simulink model "DT4H_SIMULATION_EEE"  (R2025b)
settings: Solver=ode3  StartTime=0.0  StopTime=10.0  RelTol=1e-3
libraries: simulink x19, dspstat3 x6, fuzblock x1
(part 1 of 3)
settings Model: Creator=harsh  LastModifiedBy=harsh

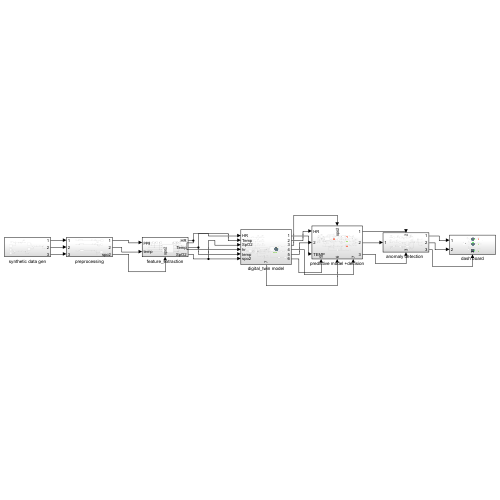
[thumbnail: Simulink's stored preview of the top-level diagram]
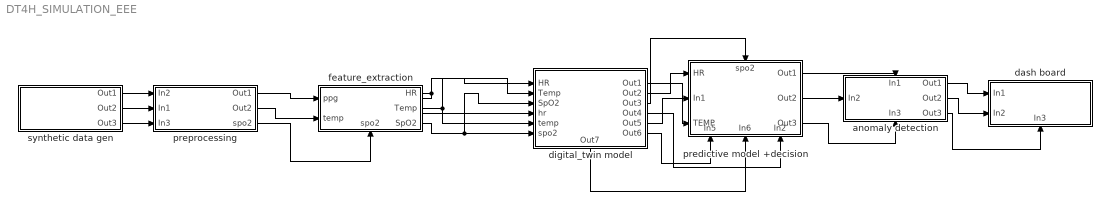
== system DT4H_SIMULATION_EEE ==
  "anomaly detection  " : Subsystem
      settings: PortSchema="{\"entries\":[{\"content\":{\"sides\":[{\"content\":{\"connectorIds\":[\"In1\"]},\"type\":\"ConnectorPlacement.EquallySpacedRectSide\",\"uuid\":\"25253e62-3c40-49ae-b2f5-e9d5db3c8bc6\"},{\"content\":{\"connectorIds\":[\"Out1\",\"Out2\",\"Out3\"],\"side\":\"RIGHT\"},\"type\":\"ConnectorPlacement.EquallySpacedRectSide\",\"uuid\":\"f4a70f19-11e9-4566-a749-a521162cf708\"},{\"content\":{\"connectorIds\":[\"In2\"],\"side\":\"TOP\"},\"type\":\"ConnectorPlacement.EquallySpacedRectSide\",\"uuid\":\"d5382edc-197f-43a2-9fdd-3d2ad96da76a\"},{\"content\":{\"connectorIds\":[\"In3\"],\"side\":\"BOTTOM\"},\"type\":\"ConnectorPlacement.EquallySpacedRectSide\",\"uuid\":\"cc34089e-1bbc-443e-9edf-3f88c550613d\"}]},\"type\":\"ConnectorPlacement.EquallySpacedConnector\",\"uuid\":\"d18f1512-da4b-4774-865f-899ab03939b9\"}],\"packageUris\":[\"http://schema.mathworks.com/mf0/Connector/R2020b\"],\"version\":\"1.0\"}"
  dash board : Subsystem
      settings: PortSchema="{\"entries\":[{\"content\":{\"sides\":[{\"content\":{\"connectorIds\":[\"In1\",\"In2\"]},\"type\":\"ConnectorPlacement.EquallySpacedRectSide\",\"uuid\":\"cdd0eb8c-e2f0-4f49-b522-7982e33a9b2a\"},{\"content\":{\"side\":\"RIGHT\"},\"type\":\"ConnectorPlacement.EquallySpacedRectSide\",\"uuid\":\"02186336-f3a8-4644-896c-78cbe002086a\"},{\"content\":{\"side\":\"TOP\"},\"type\":\"ConnectorPlacement.EquallySpacedRectSide\",\"uuid\":\"908a15e8-0b5f-4f2f-82b4-ba6efd9ebe98\"},{\"content\":{\"connectorIds\":[\"In3\"],\"side\":\"BOTTOM\"},\"type\":\"ConnectorPlacement.EquallySpacedRectSide\",\"uuid\":\"1bb7e8d6-76d1-4f36-b622-8394fe1e0f54\"}]},\"type\":\"ConnectorPlacement.EquallySpacedConnector\",\"uuid\":\"3009d2cf-5250-4716-8b2f-345bda64d323\"}],\"packageUris\":[\"http://schema.mathworks.com/mf0/Connector/R2020b\"],\"version\":\"1.0\"}"
  digital_twin model : Subsystem
      settings: PortSchema="{\"entries\":[{\"content\":{\"sides\":[{\"content\":{\"connectorIds\":[\"In1\",\"In2\",\"In3\",\"In4\",\"In5\",\"In6\"]},\"type\":\"ConnectorPlacement.EquallySpacedRectSide\",\"uuid\":\"60b3441d-3906-42cd-a64f-c568a4e10bef\"},{\"content\":{\"connectorIds\":[\"Out1\",\"Out2\",\"Out3\",\"Out4\",\"Out5\",\"Out6\"],\"side\":\"RIGHT\"},\"type\":\"ConnectorPlacement.EquallySpacedRectSide\",\"uuid\":\"87df974d-96fc-4f5d-987f-b85e09fb9cb4\"},{\"content\":{\"side\":\"TOP\"},\"type\":\"ConnectorPlacement.EquallySpacedRectSide\",\"uuid\":\"bcc1c708-069a-4209-9e3d-4d3f31c3ddac\"},{\"content\":{\"connectorIds\":[\"Out7\"],\"side\":\"BOTTOM\"},\"type\":\"ConnectorPlacement.EquallySpacedRectSide\",\"uuid\":\"6497df40-0368-42cc-9f26-60ecc793cf19\"}]},\"type\":\"ConnectorPlacement.EquallySpacedConnector\",\"uuid\":\"1b248ab8-3cfb-4c5b-9a5f-89bd9e36bb2e\"}],\"packageUris\":[\"http://schema.mathworks.com/mf0/Connector/R2020b\"],\"version\":\"1.0\"}"
  feature_extraction : Subsystem
      settings: PortSchema="{\"entries\":[{\"content\":{\"sides\":[{\"content\":{\"connectorIds\":[\"In1\",\"In2\"]},\"type\":\"ConnectorPlacement.EquallySpacedRectSide\",\"uuid\":\"0c4b2ed4-113f-4166-b962-4d2c86f0b3f8\"},{\"content\":{\"connectorIds\":[\"Out1\",\"Out2\",\"Out3\"],\"side\":\"RIGHT\"},\"type\":\"ConnectorPlacement.EquallySpacedRectSide\",\"uuid\":\"e3832425-a364-440c-8c10-9734fc320651\"},{\"content\":{\"side\":\"TOP\"},\"type\":\"ConnectorPlacement.EquallySpacedRectSide\",\"uuid\":\"36c7fb6d-317e-4b4f-ae9e-aa12a7efa738\"},{\"content\":{\"connectorIds\":[\"In3\"],\"side\":\"BOTTOM\"},\"type\":\"ConnectorPlacement.EquallySpacedRectSide\",\"uuid\":\"d821c285-c54e-4db5-b1a8-90f41e6ccbda\"}]},\"type\":\"ConnectorPlacement.EquallySpacedConnector\",\"uuid\":\"1bb0afcd-9a28-4be8-abf5-d992c306dad6\"}],\"packageUris\":[\"http://schema.mathworks.com/mf0/Connector/R2020b\"],\"version\":\"1.0\"}"
  predictive model +decision : Subsystem
      settings: PortSchema="{\"entries\":[{\"content\":{\"sides\":[{\"content\":{\"connectorIds\":[\"In1\",\"In2\",\"In3\"]},\"type\":\"ConnectorPlacement.EquallySpacedRectSide\",\"uuid\":\"b7d4fdfc-ed91-464e-87ae-7c928519d529\"},{\"content\":{\"connectorIds\":[\"Out1\",\"Out2\",\"Out3\"],\"side\":\"RIGHT\"},\"type\":\"ConnectorPlacement.EquallySpacedRectSide\",\"uuid\":\"11799bdd-7268-4954-a90f-71333eb12373\"},{\"content\":{\"connectorIds\":[\"In4\"],\"side\":\"TOP\"},\"type\":\"ConnectorPlacement.EquallySpacedRectSide\",\"uuid\":\"f3428630-4ced-4085-ba1c-f5b921f7daca\"},{\"content\":{\"connectorIds\":[\"In5\",\"In6\",\"In7\"],\"side\":\"BOTTOM\"},\"type\":\"ConnectorPlacement.EquallySpacedRectSide\",\"uuid\":\"6bf4046d-5d73-4edf-8fc4-5c2e0fba2535\"}]},\"type\":\"ConnectorPlacement.EquallySpacedConnector\",\"uuid\":\"07f606c2-3e00-4eb2-b545-ac31073d3b11\"}],\"packageUris\":[\"http://schema.mathworks.com/mf0/Connector/R2020b\"],\"version\":\"1.0\"}"
  preprocessing : Subsystem
  synthetic data gen : Subsystem
  wires:
  feature_extraction/3(SpO2) -> digital_twin model/3(SpO2), digital_twin model/6(spo2)
  digital_twin model/6(Out6) -> predictive model +decision/5(In5)
  "anomaly detection  "/2(Out2) -> dash board/2(In2)
  predictive model +decision/3(Out3) -> "anomaly detection  "/3(In3)
  feature_extraction/2(Temp) -> digital_twin model/5(temp), digital_twin model/2(Temp)
  digital_twin model/2(Out2) -> predictive model +decision/1(HR)
  preprocessing/3(spo2) -> feature_extraction/3(spo2)
  digital_twin model/3(Out3) -> predictive model +decision/4(spo2)
  digital_twin model/1(Out1) -> predictive model +decision/3(TEMP)
  digital_twin model/4(Out4) -> predictive model +decision/7(In2)
  synthetic data gen/1(Out1) -> preprocessing/1(In2)
  "anomaly detection  "/1(Out1) -> dash board/1(In1)
  predictive model +decision/1(Out1) -> "anomaly detection  "/2(In1)
  synthetic data gen/3(Out3) -> preprocessing/3(In3)
  preprocessing/1(Out1) -> feature_extraction/1(ppg)
  predictive model +decision/2(Out2) -> "anomaly detection  "/1(In2)
  digital_twin model/5(Out5) -> predictive model +decision/2(In1)
  feature_extraction/1(HR) -> digital_twin model/4(hr), digital_twin model/1(HR)
  "anomaly detection  "/3(Out3) -> dash board/3(In3)
  digital_twin model/7(Out7) -> predictive model +decision/6(In6)
  preprocessing/2(Out2) -> feature_extraction/2(temp)
  synthetic data gen/2(Out2) -> preprocessing/2(In1)

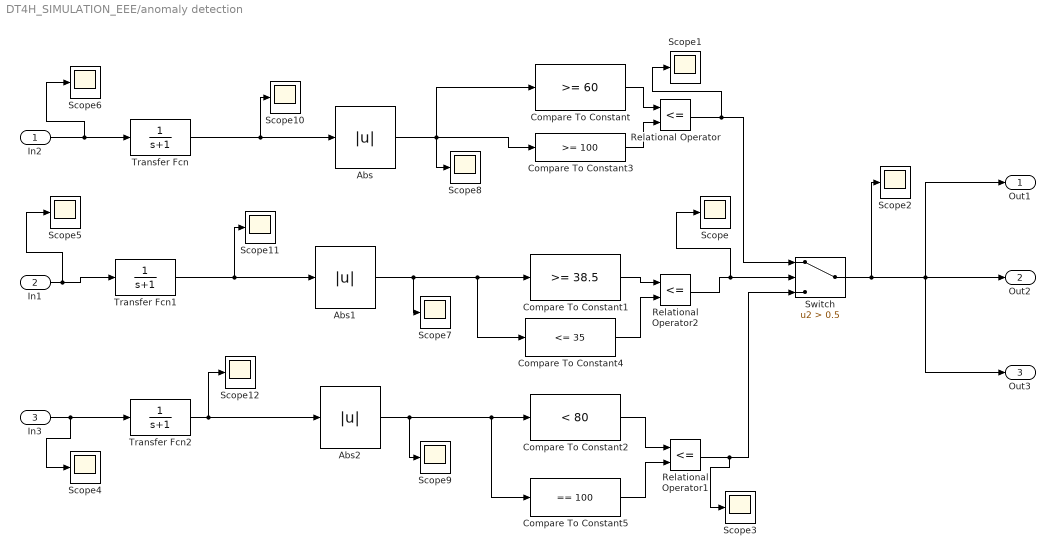
== system DT4H_SIMULATION_EEE/anomaly detection   ==
  In2 : Inport
  In1 : Inport  Port=2
  In3 : Inport  Port=3
  Abs : Abs  SaturateOnIntegerOverflow=off
  Abs1 : Abs  SaturateOnIntegerOverflow=off
  Abs2 : Abs  SaturateOnIntegerOverflow=off
  Compare To Constant : simulink/Logic and Bit Operations/Compare To Constant  relop=>=  const=60  OutDataTypeStr=boolean
  Compare To Constant1 : simulink/Logic and Bit Operations/Compare To Constant  relop=>=  const=38.5  OutDataTypeStr=boolean
  Compare To Constant2 : simulink/Logic and Bit Operations/Compare To Constant  relop=<  const=80  OutDataTypeStr=boolean
  Compare To Constant3 : simulink/Logic and Bit Operations/Compare To Constant  relop=>=  const=100  OutDataTypeStr=boolean
  Compare To Constant4 : simulink/Logic and Bit Operations/Compare To Constant  relop=<=  const=35  OutDataTypeStr=boolean
  Compare To Constant5 : simulink/Logic and Bit Operations/Compare To Constant  relop===  const=100  OutDataTypeStr=boolean
  Relational Operator : RelationalOperator  Operator=<=  OutDataTypeStr=boolean  RndMeth=Simplest  InputSameDT=off
  Relational Operator1 : RelationalOperator  Operator=<=  OutDataTypeStr=boolean  RndMeth=Simplest  InputSameDT=off
  Relational Operator2 : RelationalOperator  Operator=<=  OutDataTypeStr=boolean  RndMeth=Simplest  InputSameDT=off
  Scope{,1..12} (13 alike) : Scope
      Scope settings: ActiveDisplayYMinimum=-0.1649767287234043  ActiveDisplayYMaximum=1.1475232712765957  DataLoggingVariableName=ScopeData35  DataLoggingSaveFormat=Array
      Scope1 settings: ActiveDisplayYMinimum=-1.3578393063829792  ActiveDisplayYMaximum=1.4563615389295217  DataLoggingVariableName=ScopeData36  DataLoggingSaveFormat=Array
      Scope10 settings: ActiveDisplayYMinimum=-0.48272800637728419  ActiveDisplayYMaximum=1.3640066102669111  DataLoggingVariableName=ScopeData45  DataLoggingSaveFormat=Array
      Scope11 settings: ActiveDisplayYMinimum=-1  ActiveDisplayYMaximum=1  DataLoggingVariableName=ScopeData46  DataLoggingSaveFormat=Array
      Scope12 settings: ActiveDisplayYMinimum=-1  ActiveDisplayYMaximum=1  DataLoggingVariableName=ScopeData47  DataLoggingSaveFormat=Array
      Scope2 settings: ActiveDisplayYMinimum=-0.61808118008886315  ActiveDisplayYMaximum=1.4180371033829395  DataLoggingVariableName=ScopeData37  DataLoggingSaveFormat=Array
      Scope3 settings: ActiveDisplayYMinimum=-0.28820857928494759  ActiveDisplayYMaximum=0.38906240889493249  DataLoggingVariableName=ScopeData38  DataLoggingSaveFormat=Array
      Scope4 settings: DataLoggingVariableName=ScopeData39  DataLoggingSaveFormat=Array
      Scope5 settings: ActiveDisplayYMinimum=-1  ActiveDisplayYMaximum=1  DataLoggingVariableName=ScopeData40  DataLoggingSaveFormat=Array
      Scope6 settings: ActiveDisplayYMinimum=-0.76679867880396024  ActiveDisplayYMaximum=2.0174991785309779  DataLoggingVariableName=ScopeData41  DataLoggingSaveFormat=Array
      Scope7 settings: ActiveDisplayYMinimum=-0.0012437708333333331  ActiveDisplayYMaximum=0.011193937499999999  DataLoggingVariableName=ScopeData42  DataLoggingSaveFormat=Array
      Scope8 settings: ActiveDisplayYMinimum=-39.85588749272776  ActiveDisplayYMaximum=127.6560675853973  DataLoggingVariableName=ScopeData43  DataLoggingSaveFormat=Array
      Scope9 settings: ActiveDisplayYMinimum=-0.0015484589469588125  ActiveDisplayYMaximum=0.011511134803041187  DataLoggingVariableName=ScopeData44  DataLoggingSaveFormat=Array
  Switch : Switch  Criteria=u2 > Threshold  Threshold=0.5  SaturateOnIntegerOverflow=off  InputSameDT=off
  Transfer Fcn : TransferFcn  Denominator=[1 1]
  Transfer Fcn1 : TransferFcn  Denominator=[1 1]
  Transfer Fcn2 : TransferFcn  Denominator=[1 1]
  Out1 : Outport  VectorParamsAs1DForOutWhenUnconnected=off
  Out2 : Outport  Port=2  VectorParamsAs1DForOutWhenUnconnected=off
  Out3 : Outport  Port=3  VectorParamsAs1DForOutWhenUnconnected=off
  wires:
  Transfer Fcn/1 -> Scope10/1, Abs/1
  Abs/1 -> Compare To Constant3/1, Scope8/1, Compare To Constant/1
  In2/1 -> Transfer Fcn/1, Scope6/1
  Transfer Fcn1/1 -> Scope11/1, Abs1/1
  Abs1/1 -> Scope7/1, Compare To Constant4/1, Compare To Constant1/1
  Transfer Fcn2/1 -> Abs2/1, Scope12/1
  In1/1 -> Transfer Fcn1/1, Scope5/1
  In3/1 -> Transfer Fcn2/1, Scope4/1
  Switch/1 -> Scope2/1, Out3/1, Out2/1, Out1/1
  Compare To Constant/1 -> Relational Operator/1
  Compare To Constant3/1 -> Relational Operator/2
  Relational Operator/1 -> Scope1/1, Switch/1
  Compare To Constant2/1 -> Relational Operator1/1
  Compare To Constant5/1 -> Relational Operator1/2
  Relational Operator1/1 -> Scope3/1, Switch/3
  Compare To Constant1/1 -> Relational Operator2/1
  Compare To Constant4/1 -> Relational Operator2/2
  Relational Operator2/1 -> Scope/1, Switch/2
  Abs2/1 -> Scope9/1, Compare To Constant5/1, Compare To Constant2/1
